simulink model "sm_car_Axle3_withDSD"  (R2022a)
settings: Solver=ode23t  StartTime=0.0  StopTime=40  MaxStep=0.4  RelTol=1e-3  AbsTol=1e-3  EnableMultiTasking=on
PreLoadFcn:
  | disp('Loading default data for 3-axle vehicle and 2-axle trailer')
  | if verLessThan('matlab', '9.11')
  |     load Vehicle_Axle3_008
  |     Vehicle = Vehicle_Axle3_008;
  |     load Trailer_Axle2_000
  |     Trailer = Trailer_Axle2_000;
  | else
  |     load Vehicle_Axle3_019
  |     Vehicle = Vehicle_Axle3_019;
  |     load Trailer_Axle2_022
  |     Trailer = Trailer_Axle2_022;
  | end
  | 
  | disp('Turning off MFEval warnings...')
  | disp('Solver:CoeffChecks:Eyk -- OFF')
  | disp('Solver:Limits:Exceeded -- OFF')
  | disp('Solver:CoeffChecks:Et -- OFF')
  | disp('Solver:CoeffChecks:Exa -- OFF')
  | 
  | warning('off','Solver:CoeffChecks:Eyk')
  | warning('off','Solver:Limits:Exceeded')
  | warning('off','Solver:CoeffChecks:Et')
  | warning('off','Solver:CoeffChecks:Exa')
  | %warning('off','Solver:Radius:NegativeRho')
  | 
  | % Due to usability issue in Repeating Sequence block
  | warning('off','Simulink:Masking:Invalid');
  | 
  | % Eliminate unnecessary warnings in inactive variants
  | % Warnings generated only if you click through inactive variant
  | warning('off','MATLAB:nonExistentField');
  | warning('off','Simulink:Parameters:BlkParamUndefined');
PostLoadFcn:
  | set_param([bdroot '/Vehicle'],'popup_trailer','On')
  | warning('off','sm:sli:setup:compile:LocalSolverNotSupported')
  | sm_car_config_maneuver(bdroot,'WOT Braking');
  | sm_car_config_vehicle(bdroot,false);
  | sm_car_config_logging(bdroot);
InitFcn:
  | sm_car_config_camera;
  | Vehicle = sm_car_vehcfg_checkConfig(Vehicle);
StartFcn:
  | sm_car_check_tire_model(bdroot);
  | tic;
StopFcn:
  | Elapsed_Sim_Time = toc;
  | % disp(['Elapsed Sim Time = ' num2str(Elapsed_Sim_Time)]);
values from neighbouring files (symbols this model uses):
  scenario = drivingScenario    [AEB_PedestrianChild_Nearside_50width_overrun.m]
undefined symbols (not defined in the file or in its folder): Maneuver, SimParams, X, Y, Z
libraries: simulink x16, Tire_Utilities x7, sm_lib x6, sm_car_DSD_lib x3, World_Config_Utilities x2, Maneuver_Get_Pose x2, Vehicle_Visualization x2, drivingscenarioandsensors x1, Camera_Frame_Definitions x1, Brake_Control x1, Driveline_Control_Axle2_None x1, Power_Control_Axle2_FixedRatio x1
(part 2 of 3)

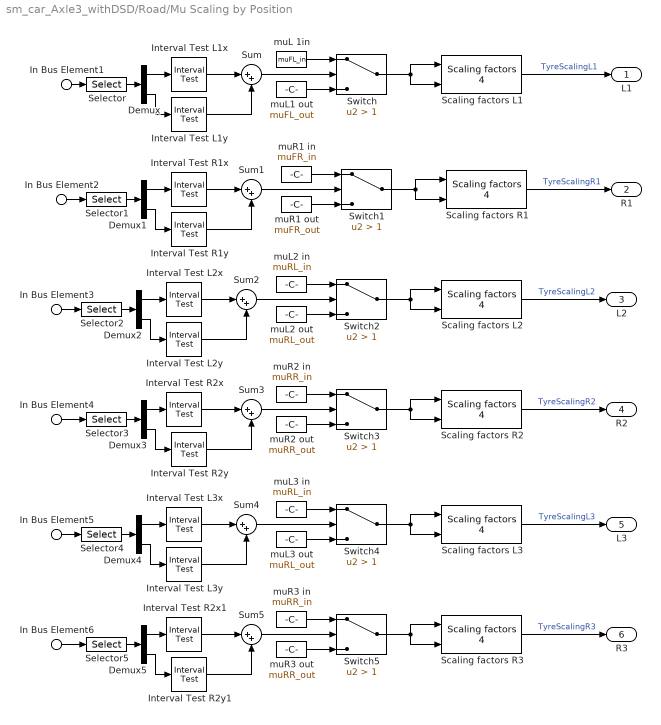
== system sm_car_Axle3_withDSD/Road/Mu Scaling by Position ==
  In Bus Element1 : Inport  PortName=Chassis  Element=WhlL1.xyz
  In Bus Element2 : Inport  PortName=Chassis  Element=WhlR1.xyz
  In Bus Element3 : Inport  PortName=Chassis  Element=WhlL2.xyz
  In Bus Element4 : Inport  PortName=Chassis  Element=WhlR2.xyz
  In Bus Element5 : Inport  PortName=Chassis  Element=WhlL3.xyz
  In Bus Element6 : Inport  PortName=Chassis  Element=WhlR3.xyz
  Demux{,1..5} (6 alike) : Demux  Outputs=2
  Interval Test L1x : simulink/Logic and Bit Operations/Interval Test  IntervalClosedRight=on  uplimit=intvX_FL_end  IntervalClosedLeft=on  lowlimit=intvX_FL_start  OutDataTypeStr=uint8
  Interval Test L1y : simulink/Logic and Bit Operations/Interval Test  IntervalClosedRight=on  uplimit=intvY_FL_end  IntervalClosedLeft=on  lowlimit=intvY_FL_start  OutDataTypeStr=uint8
  Interval Test L2x : simulink/Logic and Bit Operations/Interval Test  IntervalClosedRight=on  uplimit=intvX_RL_end  IntervalClosedLeft=on  lowlimit=intvX_RL_start  OutDataTypeStr=uint8
  Interval Test L2y : simulink/Logic and Bit Operations/Interval Test  IntervalClosedRight=on  uplimit=intvY_RL_end  IntervalClosedLeft=on  lowlimit=intvY_RL_start  OutDataTypeStr=uint8
  Interval Test L3x : simulink/Logic and Bit Operations/Interval Test  IntervalClosedRight=on  uplimit=intvX_RL_end  IntervalClosedLeft=on  lowlimit=intvX_RL_start  OutDataTypeStr=uint8
  Interval Test L3y : simulink/Logic and Bit Operations/Interval Test  IntervalClosedRight=on  uplimit=intvY_RL_end  IntervalClosedLeft=on  lowlimit=intvY_RL_start  OutDataTypeStr=uint8
  Interval Test R1x : simulink/Logic and Bit Operations/Interval Test  IntervalClosedRight=on  uplimit=intvX_FR_end  IntervalClosedLeft=on  lowlimit=intvX_FR_start  OutDataTypeStr=uint8
  Interval Test R1y : simulink/Logic and Bit Operations/Interval Test  IntervalClosedRight=on  uplimit=intvY_FR_end  IntervalClosedLeft=on  lowlimit=intvY_FR_start  OutDataTypeStr=uint8
  Interval Test R2x : simulink/Logic and Bit Operations/Interval Test  IntervalClosedRight=on  uplimit=intvX_RR_end  IntervalClosedLeft=on  lowlimit=intvX_RR_start  OutDataTypeStr=uint8
  Interval Test R2x1 : simulink/Logic and Bit Operations/Interval Test  IntervalClosedRight=on  uplimit=intvX_RR_end  IntervalClosedLeft=on  lowlimit=intvX_RR_start  OutDataTypeStr=uint8
  Interval Test R2y : simulink/Logic and Bit Operations/Interval Test  IntervalClosedRight=on  uplimit=intvY_RR_end  IntervalClosedLeft=on  lowlimit=intvY_RR_start  OutDataTypeStr=uint8
  Interval Test R2y1 : simulink/Logic and Bit Operations/Interval Test  IntervalClosedRight=on  uplimit=intvY_RR_end  IntervalClosedLeft=on  lowlimit=intvY_RR_start  OutDataTypeStr=uint8
  Scaling factors L1 : Tire_Utilities/Scaling factors 4  LKX=1  LKY=1  LKYC=1  LTR=1  LKZC=1
  Scaling factors L2 : Tire_Utilities/Scaling factors 4  LKX=1  LKY=1  LKYC=1  LTR=1  LKZC=1
  Scaling factors L3 : Tire_Utilities/Scaling factors 4  LKX=1  LKY=1  LKYC=1  LTR=1  LKZC=1
  Scaling factors R1 : Tire_Utilities/Scaling factors 4  LKX=1  LKY=1  LKYC=1  LTR=1  LKZC=1
  Scaling factors R2 : Tire_Utilities/Scaling factors 4  LKX=1  LKY=1  LKYC=1  LTR=1  LKZC=1
  Scaling factors R3 : Tire_Utilities/Scaling factors 4  LKX=1  LKY=1  LKYC=1  LTR=1  LKZC=1
  Selector{,1..5} (6 alike) : Selector  InputPortWidth=3  IndexOptions=Index vector (dialog)  Indices=[1 2]  OutputSizes=1
  Sum{,1..5} (6 alike) : Sum  Inputs=|++
  Switch : Switch  Criteria=u2 > Threshold  Threshold=1  ZeroCross=off  SaturateOnIntegerOverflow=off  InputSameDT=off
  Switch{1..5} (5 alike) : Switch  Criteria=u2 > Threshold  Threshold=1  SaturateOnIntegerOverflow=off  InputSameDT=off
  muL 1in : Constant  Value=muFL_in
  muL1 out : Constant  Value=muFL_out
  muL2 in : Constant  Value=muRL_in
  muL2 out : Constant  Value=muRL_out
  muL3 in : Constant  Value=muRL_in
  muL3 out : Constant  Value=muRL_out
  muR1 in : Constant  Value=muFR_in
  muR1 out : Constant  Value=muFR_out
  muR2 in : Constant  Value=muRR_in
  muR2 out : Constant  Value=muRR_out
  muR3 in : Constant  Value=muRR_in
  muR3 out : Constant  Value=muRR_out
  L1 : Outport  VectorParamsAs1DForOutWhenUnconnected=off
  R1 : Outport  Port=2  VectorParamsAs1DForOutWhenUnconnected=off
  L2 : Outport  Port=3  VectorParamsAs1DForOutWhenUnconnected=off
  R2 : Outport  Port=4  VectorParamsAs1DForOutWhenUnconnected=off
  L3 : Outport  Port=5  VectorParamsAs1DForOutWhenUnconnected=off
  R3 : Outport  Port=6  VectorParamsAs1DForOutWhenUnconnected=off
  wires:
  Demux/1 -> Interval Test L1x/1
  Interval Test R2x/1 -> Sum3/1
  Demux3/2 -> Interval Test R2y/1
  Demux3/1 -> Interval Test R2x/1
  Sum3/1 -> Switch3/2
  Selector3/1 -> Demux3/1
  In Bus Element4/1 -> Selector3/1
  Interval Test R2y/1 -> Sum3/2
  Demux2/2 -> Interval Test L2y/1
  Selector2/1 -> Demux2/1
  Demux2/1 -> Interval Test L2x/1
  Interval Test L2y/1 -> Sum2/2
  Sum2/1 -> Switch2/2
  In Bus Element3/1 -> Selector2/1
  Interval Test L2x/1 -> Sum2/1
  Interval Test R1y/1 -> Sum1/2
  Selector1/1 -> Demux1/1
  Demux1/2 -> Interval Test R1y/1
  Sum1/1 -> Switch1/2
  Demux1/1 -> Interval Test R1x/1
  Interval Test R1x/1 -> Sum1/1
  Interval Test L1x/1 -> Sum/1
  Interval Test L1y/1 -> Sum/2
  Sum/1 -> Switch/2
  Demux/2 -> Interval Test L1y/1
  Selector/1 -> Demux/1
  muR2 out/1 -> Switch3/3
  muR2 in/1 -> Switch3/1
  Switch3/1 -> Scaling factors R2/2, Scaling factors R2/1
  Scaling factors R2/1 -> R2/1  "TyreScalingR2"
  Scaling factors L2/1 -> L2/1  "TyreScalingL2"
  Switch2/1 -> Scaling factors L2/1, Scaling factors L2/2
  muL2 in/1 -> Switch2/1
  muL2 out/1 -> Switch2/3
  muR1 out/1 -> Switch1/3
  In Bus Element2/1 -> Selector1/1
  muR1 in/1 -> Switch1/1
  Switch1/1 -> Scaling factors R1/2, Scaling factors R1/1
  Scaling factors R1/1 -> R1/1  "TyreScalingR1"
  Scaling factors L1/1 -> L1/1  "TyreScalingL1"
  Switch/1 -> Scaling factors L1/1, Scaling factors L1/2
  muL1 out/1 -> Switch/3
  muL 1in/1 -> Switch/1
  In Bus Element1/1 -> Selector/1
  muL3 out/1 -> Switch4/3
  Switch4/1 -> Scaling factors L3/2, Scaling factors L3/1
  Scaling factors L3/1 -> L3/1  "TyreScalingL3"
  Scaling factors R3/1 -> R3/1  "TyreScalingR3"
  Switch5/1 -> Scaling factors R3/1, Scaling factors R3/2
  muR3 in/1 -> Switch5/1
  muR3 out/1 -> Switch5/3
  Interval Test L3x/1 -> Sum4/1
  In Bus Element5/1 -> Selector4/1
  Sum4/1 -> Switch4/2
  Interval Test L3y/1 -> Sum4/2
  Demux4/1 -> Interval Test L3x/1
  Selector4/1 -> Demux4/1
  Demux4/2 -> Interval Test L3y/1
  Interval Test R2y1/1 -> Sum5/2
  In Bus Element6/1 -> Selector5/1
  Selector5/1 -> Demux5/1
  Sum5/1 -> Switch5/2
  Demux5/1 -> Interval Test R2x1/1
  Demux5/2 -> Interval Test R2y1/1
  Interval Test R2x1/1 -> Sum5/1
  muL3 in/1 -> Switch4/1

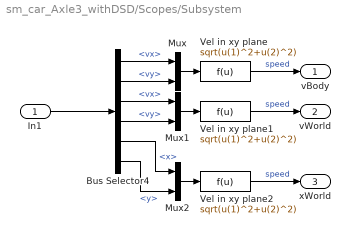
== system sm_car_Axle3_withDSD/Scopes/Subsystem ==
  In1 : Inport
  Bus Selector4 : BusSelector  OutputSignals=Chassis.Body.CG.vx,Chassis.Body.CG.vy,World.vx,World.vy,World.x,World.y
  Mux : Mux  Inputs=2
  Mux1 : Mux  Inputs=2
  Mux2 : Mux  Inputs=2
  Vel in xy plane : Fcn  Expr=sqrt(u(1)^2+u(2)^2)
  Vel in xy plane1 : Fcn  Expr=sqrt(u(1)^2+u(2)^2)
  Vel in xy plane2 : Fcn  Expr=sqrt(u(1)^2+u(2)^2)
  vBody : Outport  VectorParamsAs1DForOutWhenUnconnected=off
  vWorld : Outport  Port=2  VectorParamsAs1DForOutWhenUnconnected=off
  xWorld : Outport  Port=3  VectorParamsAs1DForOutWhenUnconnected=off
  wires:
  Bus Selector4/3 -> Mux1/1  "<vx>"
  Bus Selector4/4 -> Mux1/2  "<vy>"
  Bus Selector4/1 -> Mux/1  "<vx>"
  Vel in xy plane1/1 -> vWorld/1  "speed"
  In1/1 -> Bus Selector4/1
  Mux1/1 -> Vel in xy plane1/1
  Mux/1 -> Vel in xy plane/1
  Vel in xy plane/1 -> vBody/1  "speed"
  Bus Selector4/2 -> Mux/2  "<vy>"
  Mux2/1 -> Vel in xy plane2/1
  Bus Selector4/6 -> Mux2/2  "<y>"
  Bus Selector4/5 -> Mux2/1  "<x>"
  Vel in xy plane2/1 -> xWorld/1  "speed"

== system sm_car_Axle3_withDSD/Vehicle/Hitch ==
  Off : Subsystem  VariantControl=Off
  On : Subsystem  VariantControl=On
  " F" : PMIOPort  Side=Right
  " B" : PMIOPort  Port=2  Side=Left

== system sm_car_Axle3_withDSD/Vehicle/Vehicle Constraint ==
  No Constraint : Subsystem  VariantControl=NoConstraint
  No Yaw : Subsystem  VariantControl=NoYaw
  F : PMIOPort  Side=Right
  B : PMIOPort  Port=2  Side=Left

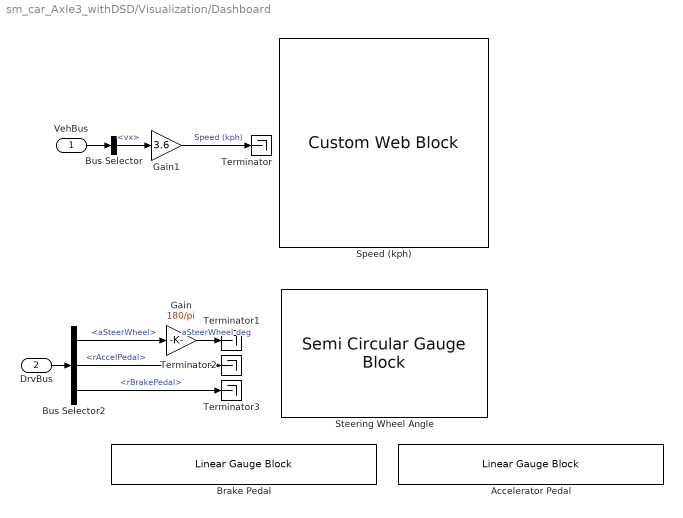
== system sm_car_Axle3_withDSD/Visualization/Dashboard ==
  VehBus : Inport
  DrvBus : Inport  Port=2
  Accelerator Pedal : LinearGaugeBlock  LabelPosition=Hide  ScaleMax=1
  Brake Pedal : LinearGaugeBlock  ScaleMax=1
  Bus Selector : BusSelector  OutputSignals=Chassis.Body.CG.vx
  Bus Selector2 : BusSelector  OutputSignals=aSteerWheel,rAccelPedal,rBrakePedal
  Gain : Gain  Gain=180/pi
  Gain1 : Gain  Gain=3.6
  Speed (kph) : CustomWebBlock  LabelPosition=Hide  ShowInitialText=on  Configuration="{\"components\":[{\"name\":\"CircularScaleComponent\",\"settings\":{\"bounds\":{\"max\":150,\"min\":0,\"tickInterval\":\"auto\"},\"direction\":\"cw\",\"flipLimits\":0,\"innerRadius\":0.46396628518311167,\"internalTickHeightScaleFactor\":1,\"labelColor\":[250,245,200],\"labelFont\":{\"font\":\"Arial\",\"fontSize\":12},\"labelRadius\":0.3050476634899135,\"labelTransparency\":1,\"minorTickHeightScaleFactor\":0.2,\"needleImage\":{\"size\":[1890,567],\"src\":\"data:image\\/svg+xml;base64,PD94bWwgdmVyc2lvbj0iMS4wIiBlbmNvZGluZz0iVVRGLTgiIHN0YW5kYWxvbmU9Im5vIj8+CjxzdmcKICAgeG1sbnM6ZGM9Imh0dHA6Ly9wdXJsLm9yZy9kYy9lbGVtZW50cy8xLjEvIgogICB4bWxuczpjYz0iaHR0cDovL2NyZWF0aXZlY29tbW9ucy5vcmcvbnMjIgogICB4bWxuczpyZGY9Imh0dHA6Ly93d3cudzMub3JnLzE5OTkvMDIvMjItcmRmLXN5bnRheC1ucyMiCiAgIHhtbG5zOnN2Zz0iaHR0cDovL3d3dy53My5vcmcvMjAwMC9zdmciCiAgIHhtbG5zPSJodHRwOi8vd3d3LnczLm9yZy8yMDAwL3N2ZyIKICAgeG1sbnM6 ...(+4096 chars)\"},\"needleOffset\":[0.09689320773631488,0],\"needleOrientation\":-45,\"needleRotation\":-180,\"needleSize\":{\"height\":0.0899722643265781,\"width\":0.2837586797992078},\"outerRadius\":0.6228849068763098,\"position\":[0,0,1,1],\"referencePoint\":\"auto\",\"scaleAngle\":299.999999999988,\"scaleAngleOffset\":119.46147497096791,\"scaleColors\":[],\"scaleColorsSize\":0.2,\"scaleDirection\":\"CW\",\"scalePosition\":[0,0,1,1],\"showLabels\":1,\"showMinorTicks\":1,\"showSpanLine\":1,\"showTicks\":1,\"tickColor\":[250,245,200],\"tickTransparency\":1,\"valueBarColor\":[23,89,176],\"valueBarPosition\":[0,0,1,1],\"valueBarSize\":0.2,\"valueBarTransparency\":1}},{\"name\":\"BackgroundImageComponent\",\"settings\":{\"image\":{\"size\":[0,0],\"src\":\"data:image\\/svg+xml;base64,PD94bWwgdmVyc2lvbj0iMS4wIiBlbmNvZGluZz0iVVRGLTgiIHN0YW5kYWxvbmU9Im5vIj8+CjwhLS0gR2VuZXJhdG9yOiBBZG9iZSBJbGx1c3RyYXRvciAxOS4yLjEsIFNWRyBFeHBvcnQgUGx1Zy1JbiAuIFNWRyBWZXJzaW9uOiA2LjAwIEJ1aWxkIDApICAtLT4KCjxzdmcKICAgeG1sbnM6ZGM9Imh0dHA6Ly9wdXJsLm9yZy9kYy9lbGVtZW50cy8xLjEvIgogICB4bWxuczpjYz0iaHR0cDovL2NyZWF0aXZlY29tbW9ucy5vcmcvbnMjIgogICB4bWxuczpyZGY9Imh0dHA6Ly93d3cudzMub3JnLzE5OTkvMDIvMjItcmRmLXN5bnRh ...(+9660 chars)\",\"srcOrientation\":\"horizontal\"},\"position\":[0,0,1,1],\"scaleMode\":\"0\"}},{\"name\":\"ForegroundImageComponent\",\"settings\":{\"image\":{\"size\":[0,0],\"src\":\"default\",\"srcOrientation\":[]},\"isForeground\":1,\"position\":[0,0,1,1],\"scaleMode\":\"0\"}}],\"settings\":{\"BindingType\":\"signal\",\"backgroundOffset\":0.14,\"backgroundOpacity\":1,\"fixedAspectRatio\":\"on\",\"orientation\":\"horizontal\",\"showBackgroundColor\":0,\"version\":\"R2022a\"},\"type\":\"CircularGauge\"}"
  Steering Wheel Angle : SemiCircularGaugeBlock  LabelPosition=Hide  ScaleMin=-80  ScaleMax=80  TickInterval=20
  Terminator{,1..3} (4 alike) : Terminator
  wires:
  VehBus/1 -> Bus Selector/1
  DrvBus/1 -> Bus Selector2/1
  Bus Selector/1 -> Gain1/1  "<vx>"
  Gain/1 -> Terminator1/1  "aSteerWheel deg"
  Bus Selector2/3 -> Terminator3/1  "<rBrakePedal>"
  Bus Selector2/1 -> Gain/1  "<aSteerWheel>"
  Bus Selector2/2 -> Terminator2/1  "<rAccelPedal>"
  Gain1/1 -> Terminator/1  "Speed (kph)"

== system sm_car_Axle3_withDSD/Visualization/Unreal ==
  "xyz " : Inport
  "rpy " : Inport  Port=2
  "ws " : Inport  Port=3
  "aCamber " : Inport  Port=4
  "aSteerWheel " : Inport  Port=5
  Animation Off : Subsystem  VariantControl=Off
  Animation On : Subsystem  VariantControl=On

== system sm_car_Axle3_withDSD/Driver/Closed Loop/Driver Override ==
  In : Inport
  None : Subsystem  VariantControl=None
  Override : Subsystem  VariantControl=Override
  DrvBus : Outport

== system sm_car_Axle3_withDSD/Driver/Closed Loop/Scopes ==
  <vx> : Inport
  Ref : Inport  Port=2
  CurPose : Inport  Port=3
  DrvBus : Inport  Port=4
  Bus Selector : BusSelector  OutputSignals=vTarget
  Bus Selector1 : BusSelector  OutputSignals=aSteerWheel,rAccelPedal,rBrakePedal
  Compare vx to Target : Scope  NumInputPorts=2
  RefPose : Scope
  Scope1 : Scope  NumInputPorts=3
  wires:
  DrvBus/1 -> Bus Selector1/1
  Bus Selector1/1 -> Scope1/1  "<aSteerWheel>"
  Bus Selector1/2 -> Scope1/2  "<rAccelPedal>"
  <vx>/1 -> Compare vx to Target/1
  Bus Selector1/3 -> Scope1/3  "<rBrakePedal>"
  CurPose/1 -> RefPose/1
  Bus Selector/1 -> Compare vx to Target/2  "<vTarget>"
  Ref/1 -> Bus Selector/1

== system sm_car_Axle3_withDSD/Driver/Interactive/Pace Car ==
  "VehBus " : Inport
  None : Subsystem  VariantControl=None
  Show : Subsystem  VariantControl=Show

== system sm_car_Axle3_withDSD/Vehicle/Hitch/Off ==
  Reference Frame : sm_lib/Frames and Transforms/Reference Frame
  F : PMIOPort  Side=Right
  B : PMIOPort  Port=2  Side=Left
  connections:
  B/RConn1 -- Reference Frame/RConn1

== system sm_car_Axle3_withDSD/Vehicle/Hitch/On ==
  Gimbal Joint : sm_lib/Joints/Gimbal Joint  JointMode=Normal  SenseConstraintForce=off  SenseConstraintForceX=off  SenseConstraintForceY=off  SenseConstraintForceZ=off  SenseConstraintTorque=off  SenseConstraintTorqueX=off  SenseConstraintTorqueY=off  SenseConstraintTorqueZ=off  SenseTotalForce=off  SenseTotalForceX=off  SenseTotalForceY=off  SenseTotalForceZ=off  SenseTotalTorque=off  SenseTotalTorqueX=off  SenseTotalTorqueY=off  SenseTotalTorqueZ=off  CompositeWrenchDir=FollowerOnBase  CompositeWrenchFrame=BaseFrame  RxEquilibriumPosition=0  RxEquilibriumPositionUnits=deg  RxSpringStiffness=1000  RxSpringStiffnessUnits=N*m/deg  RxDampingCoefficient=10  RxDampingCoefficientUnits=N*m/(deg/s)  RxTorqueActuationMode=NoTorque  RxMotionActuationMode=ComputedMotion  RxSensePosition=off  RxSenseVelocity=off  RxSenseAcceleration=off  RxSenseTorqueForce=off  RxSenseLowerLimitTorqueForce=off  RxSenseUpperLimitTorqueForce=off  RxLowerLimitSpecify=off  RxLowerLimitBound=-90  RxLowerLimitBoundUnits=deg  RxLowerLimitStiffness=1e4  RxLowerLimitStiffnessUnits=N*m/deg  RxLowerLimitDamping=10  RxLowerLimitDampingUnits=N*m/(deg/s)  RxLowerLimitTransitionRegionWidth=0.1  RxLowerLimitTransitionRegionWidthUnits=deg  RxUpperLimitSpecify=off  RxUpperLimitBound=90  RxUpperLimitBoundUnits=deg  RxUpperLimitStiffness=1e4  RxUpperLimitStiffnessUnits=N*m/deg  RxUpperLimitDamping=10  RxUpperLimitDampingUnits=N*m/(deg/s)  RxUpperLimitTransitionRegionWidth=0.1  RxUpperLimitTransitionRegionWidthUnits=deg  RxPositionTargetSpecify=on  RxPositionTargetPriority=High  RxPositionTargetValue=0  RxPositionTargetValueUnits=deg  RxVelocityTargetSpecify=off  RxVelocityTargetPriority=High  RxVelocityTargetValue=0  RxVelocityTargetValueUnits=deg/s  RyEquilibriumPosition=0  RyEquilibriumPositionUnits=deg  RySpringStiffness=1000  RySpringStiffnessUnits=N*m/deg  RyDampingCoefficient=10  RyDampingCoefficientUnits=N*m/(deg/s)  RyTorqueActuationMode=NoTorque  RyMotionActuationMode=ComputedMotion  RySensePosition=off  RySenseVelocity=off  RySenseAcceleration=off  RySenseTorqueForce=off  RySenseLowerLimitTorqueForce=off  RySenseUpperLimitTorqueForce=off  RyLowerLimitSpecify=off  RyLowerLimitBound=-90  RyLowerLimitBoundUnits=deg  RyLowerLimitStiffness=1e4  RyLowerLimitStiffnessUnits=N*m/deg  RyLowerLimitDamping=10  RyLowerLimitDampingUnits=N*m/(deg/s)  RyLowerLimitTransitionRegionWidth=0.1  RyLowerLimitTransitionRegionWidthUnits=deg  RyUpperLimitSpecify=off  RyUpperLimitBound=90  RyUpperLimitBoundUnits=deg  RyUpperLimitStiffness=1e4  RyUpperLimitStiffnessUnits=N*m/deg  RyUpperLimitDamping=10  RyUpperLimitDampingUnits=N*m/(deg/s)  RyUpperLimitTransitionRegionWidth=0.1  RyUpperLimitTransitionRegionWidthUnits=deg  RyPositionTargetSpecify=on  RyPositionTargetPriority=High  RyPositionTargetValue=0  RyPositionTargetValueUnits=deg  RyVelocityTargetSpecify=off  RyVelocityTargetPriority=High  RyVelocityTargetValue=0  RyVelocityTargetValueUnits=deg/s  RzEquilibriumPosition=0  RzEquilibriumPositionUnits=deg  RzSpringStiffness=0  RzSpringStiffnessUnits=N*m/deg  RzDampingCoefficient=0  RzDampingCoefficientUnits=N*m/(deg/s)  RzTorqueActuationMode=NoTorque  RzMotionActuationMode=ComputedMotion  RzSensePosition=off  RzSenseVelocity=off  RzSenseAcceleration=off  RzSenseTorqueForce=off  RzSenseLowerLimitTorqueForce=off  RzSenseUpperLimitTorqueForce=off  RzLowerLimitSpecify=off  RzLowerLimitBound=-90  RzLowerLimitBoundUnits=deg  RzLowerLimitStiffness=1e4  RzLowerLimitStiffnessUnits=N*m/deg  RzLowerLimitDamping=10  RzLowerLimitDampingUnits=N*m/(deg/s)  RzLowerLimitTransitionRegionWidth=0.1  RzLowerLimitTransitionRegionWidthUnits=deg  RzUpperLimitSpecify=off  RzUpperLimitBound=90  RzUpperLimitBoundUnits=deg  RzUpperLimitStiffness=1e4  RzUpperLimitStiffnessUnits=N*m/deg  RzUpperLimitDamping=10  RzUpperLimitDampingUnits=N*m/(deg/s)  RzUpperLimitTransitionRegionWidth=0.1  RzUpperLimitTransitionRegionWidthUnits=deg  RzPositionTargetSpecify=on  RzPositionTargetPriority=High  RzPositionTargetValue=0  RzPositionTargetValueUnits=deg  RzVelocityTargetSpecify=off  RzVelocityTargetPriority=High  RzVelocityTargetValue=0  RzVelocityTargetValueUnits=deg/s
  Spherical Joint : sm_lib/Joints/Spherical Joint  Commented=on  JointMode=Normal  SenseConstraintForce=off  SenseConstraintForceX=off  SenseConstraintForceY=off  SenseConstraintForceZ=off  SenseConstraintTorque=off  SenseConstraintTorqueX=off  SenseConstraintTorqueY=off  SenseConstraintTorqueZ=off  SenseTotalForce=off  SenseTotalForceX=off  SenseTotalForceY=off  SenseTotalForceZ=off  SenseTotalTorque=off  SenseTotalTorqueX=off  SenseTotalTorqueY=off  SenseTotalTorqueZ=off  CompositeWrenchDir=FollowerOnBase  CompositeWrenchFrame=BaseFrame  DefPosRotationMethod=None  DefPosRotationAngleUnits=deg  DefPosRotationStandardAxis=+Z  DefPosRotationAngle=0.0  DefPosRotationArbitraryAxis=[0 0 1]  DefPosFollAlignAxisA=+X  DefPosBaseAlignAxisA=+Y  DefPosFollAlignAxisB=+Y  DefPosBaseAlignAxisB=+Z  DefPosRotationSequenceAxes=FollowerAxes  DefPosRotationSequence=XYX  DefPosRotationSequenceAngles=[0 0 0]  DefPosRotationSequenceAnglesUnits=deg  DefPosRotationMatrix=[1 0 0; 0 1 0; 0 0 1]  EqPosRotationMethod=None  EqPosRotationAngleUnits=deg  EqPosRotationStandardAxis=+Z  EqPosRotationAngle=0.0  EqPosRotationArbitraryAxis=[0 0 1]  EqPosFollAlignAxisA=+X  EqPosBaseAlignAxisA=+Y  EqPosFollAlignAxisB=+Y  EqPosBaseAlignAxisB=+Z  EqPosRotationSequenceAxes=FollowerAxes  EqPosRotationSequence=XYX  EqPosRotationSequenceAngles=[0 0 0]  EqPosRotationSequenceAnglesUnits=deg  EqPosRotationMatrix=[1 0 0; 0 1 0; 0 0 1]  SpringStiffness=100  SpringStiffnessUnits=N*m/deg  DampingCoefficient=0.1  DampingCoefficientUnits=N*m/(deg/s)  ActuateTorqueX=off  ActuateTorqueY=off  ActuateTorqueZ=off  ActuateTorque=off  TorqueActuationMode=NoTorque  MotionActuationMode=ComputedMotion  ActuationFrame=BaseFrame  SensePosition=off  SenseVelocityX=off  SenseVelocityY=off  SenseVelocityZ=off  SenseVelocity=off  SenseAccelerationX=off  SenseAccelerationY=off  SenseAccelerationZ=off  SenseAcceleration=off  SenseTorqueX=off  SenseTorqueY=off  SenseTorqueZ=off  SenseTorqueForce=off  SenseLowerLimitTorqueMag=off  SenseUpperLimitTorqueMag=off  SensingFrame=BaseFrame  LowerLimitSpecify=off  LowerLimitBound=15  LowerLimitBoundUnits=deg  LowerLimitStiffness=1e4  LowerLimitStiffnessUnits=N*m/deg  LowerLimitDamping=10  LowerLimitDampingUnits=N*m/(deg/s)  LowerLimitTransitionRegionWidth=0.1  LowerLimitTransitionRegionWidthUnits=deg  UpperLimitSpecify=off  UpperLimitBound=45  UpperLimitBoundUnits=deg  UpperLimitStiffness=1e4  UpperLimitStiffnessUnits=N*m/deg  UpperLimitDamping=10  UpperLimitDampingUnits=N*m/(deg/s)  UpperLimitTransitionRegionWidth=0.1  UpperLimitTransitionRegionWidthUnits=deg  PositionTargetRotationMethod=None  PositionTargetRotationAngleUnits=deg  PositionTargetRotationStandardAxis=+Z  PositionTargetRotationAngle=0.0  PositionTargetRotationArbitraryAxis=[0 0 1]  PositionTargetFollAlignAxisA=+X  PositionTargetBaseAlignAxisA=+Y  PositionTargetFollAlignAxisB=+Y  PositionTargetBaseAlignAxisB=+Z  PositionTargetRotationSequenceAxes=FollowerAxes  PositionTargetRotationSequence=XYX  PositionTargetRotationSequenceAngles=[0 0 0]  PositionTargetRotationSequenceAnglesUnits=deg  PositionTargetRotationMatrix=[1 0 0; 0 1 0; 0 0 1]  PositionTargetSpecify=on  PositionTargetPriority=High  VelocityTargetValue=[0 0 0]  VelocityTargetValueUnits=deg/s  VelocityTargetSpecify=off  VelocityTargetPriority=High  VelocityTargetInFollowerFrame=on
  F : PMIOPort  Side=Right
  B : PMIOPort  Port=2  Side=Left
  connections:
  Gimbal Joint/LConn1 -- B/RConn1
  Gimbal Joint/RConn1 -- F/RConn1

== system sm_car_Axle3_withDSD/Vehicle/Vehicle Constraint/No Constraint ==
  F : PMIOPort  Side=Right
  B : PMIOPort  Port=2  Side=Left

== system sm_car_Axle3_withDSD/Vehicle/Vehicle Constraint/No Yaw ==
  Cartesian Joint : sm_lib/Joints/Cartesian Joint  JointMode=Normal  SenseConstraintForce=off  SenseConstraintForceX=off  SenseConstraintForceY=off  SenseConstraintForceZ=off  SenseConstraintTorque=off  SenseConstraintTorqueX=off  SenseConstraintTorqueY=off  SenseConstraintTorqueZ=off  SenseTotalForce=off  SenseTotalForceX=off  SenseTotalForceY=off  SenseTotalForceZ=off  SenseTotalTorque=off  SenseTotalTorqueX=off  SenseTotalTorqueY=off  SenseTotalTorqueZ=off  CompositeWrenchDir=FollowerOnBase  CompositeWrenchFrame=BaseFrame  PxEquilibriumPosition=0  PxEquilibriumPositionUnits=m  PxSpringStiffness=0  PxSpringStiffnessUnits=N/m  PxDampingCoefficient=0  PxDampingCoefficientUnits=N/(m/s)  PxTorqueActuationMode=NoTorque  PxMotionActuationMode=ComputedMotion  PxSensePosition=off  PxSenseVelocity=off  PxSenseAcceleration=off  PxSenseTorqueForce=off  PxSenseLowerLimitTorqueForce=off  PxSenseUpperLimitTorqueForce=off  PxLowerLimitSpecify=off  PxLowerLimitBound=-1  PxLowerLimitBoundUnits=m  PxLowerLimitStiffness=1e6  PxLowerLimitStiffnessUnits=N/m  PxLowerLimitDamping=1e3  PxLowerLimitDampingUnits=N/(m/s)  PxLowerLimitTransitionRegionWidth=1e-4  PxLowerLimitTransitionRegionWidthUnits=m  PxUpperLimitSpecify=off  PxUpperLimitBound=1  PxUpperLimitBoundUnits=m  PxUpperLimitStiffness=1e6  PxUpperLimitStiffnessUnits=N/m  PxUpperLimitDamping=1e3  PxUpperLimitDampingUnits=N/(m/s)  PxUpperLimitTransitionRegionWidth=1e-4  PxUpperLimitTransitionRegionWidthUnits=m  PxPositionTargetSpecify=off  PxPositionTargetPriority=High  PxPositionTargetValue=0  PxPositionTargetValueUnits=m  PxVelocityTargetSpecify=off  PxVelocityTargetPriority=High  PxVelocityTargetValue=0  PxVelocityTargetValueUnits=m/s  PyEquilibriumPosition=0  PyEquilibriumPositionUnits=m  PySpringStiffness=0  PySpringStiffnessUnits=N/m  PyDampingCoefficient=0  PyDampingCoefficientUnits=N/(m/s)  PyTorqueActuationMode=NoTorque  PyMotionActuationMode=ComputedMotion  PySensePosition=off  PySenseVelocity=off  PySenseAcceleration=off  PySenseTorqueForce=off  PySenseLowerLimitTorqueForce=off  PySenseUpperLimitTorqueForce=off  PyLowerLimitSpecify=off  PyLowerLimitBound=-1  PyLowerLimitBoundUnits=m  PyLowerLimitStiffness=1e6  PyLowerLimitStiffnessUnits=N/m  PyLowerLimitDamping=1e3  PyLowerLimitDampingUnits=N/(m/s)  PyLowerLimitTransitionRegionWidth=1e-4  PyLowerLimitTransitionRegionWidthUnits=m  PyUpperLimitSpecify=off  PyUpperLimitBound=1  PyUpperLimitBoundUnits=m  PyUpperLimitStiffness=1e6  PyUpperLimitStiffnessUnits=N/m  PyUpperLimitDamping=1e3  PyUpperLimitDampingUnits=N/(m/s)  PyUpperLimitTransitionRegionWidth=1e-4  PyUpperLimitTransitionRegionWidthUnits=m  PyPositionTargetSpecify=off  PyPositionTargetPriority=High  PyPositionTargetValue=0  PyPositionTargetValueUnits=m  PyVelocityTargetSpecify=off  PyVelocityTargetPriority=High  PyVelocityTargetValue=0  PyVelocityTargetValueUnits=m/s  PzEquilibriumPosition=0  PzEquilibriumPositionUnits=m  PzSpringStiffness=0  PzSpringStiffnessUnits=N/m  PzDampingCoefficient=0  PzDampingCoefficientUnits=N/(m/s)  PzTorqueActuationMode=NoTorque  PzMotionActuationMode=ComputedMotion  PzSensePosition=off  PzSenseVelocity=off  PzSenseAcceleration=off  PzSenseTorqueForce=off  PzSenseLowerLimitTorqueForce=off  PzSenseUpperLimitTorqueForce=off  PzLowerLimitSpecify=off  PzLowerLimitBound=-1  PzLowerLimitBoundUnits=m  PzLowerLimitStiffness=1e6  PzLowerLimitStiffnessUnits=N/m  PzLowerLimitDamping=1e3  PzLowerLimitDampingUnits=N/(m/s)  PzLowerLimitTransitionRegionWidth=1e-4  PzLowerLimitTransitionRegionWidthUnits=m  PzUpperLimitSpecify=off  PzUpperLimitBound=1  PzUpperLimitBoundUnits=m  PzUpperLimitStiffness=1e6  PzUpperLimitStiffnessUnits=N/m  PzUpperLimitDamping=1e3  PzUpperLimitDampingUnits=N/(m/s)  PzUpperLimitTransitionRegionWidth=1e-4  PzUpperLimitTransitionRegionWidthUnits=m  PzPositionTargetSpecify=off  PzPositionTargetPriority=High  PzPositionTargetValue=0  PzPositionTargetValueUnits=m  PzVelocityTargetSpecify=off  PzVelocityTargetPriority=High  PzVelocityTargetValue=0  PzVelocityTargetValueUnits=m/s
  Universal Joint : sm_lib/Joints/Universal Joint  JointMode=Normal  SenseConstraintForce=off  SenseConstraintForceX=off  SenseConstraintForceY=off  SenseConstraintForceZ=off  SenseConstraintTorque=off  SenseConstraintTorqueX=off  SenseConstraintTorqueY=off  SenseConstraintTorqueZ=off  SenseTotalForce=off  SenseTotalForceX=off  SenseTotalForceY=off  SenseTotalForceZ=off  SenseTotalTorque=off  SenseTotalTorqueX=off  SenseTotalTorqueY=off  SenseTotalTorqueZ=off  CompositeWrenchDir=FollowerOnBase  CompositeWrenchFrame=BaseFrame  RxEquilibriumPosition=0  RxEquilibriumPositionUnits=deg  RxSpringStiffness=0  RxSpringStiffnessUnits=N*m/deg  RxDampingCoefficient=0  RxDampingCoefficientUnits=N*m/(deg/s)  RxTorqueActuationMode=NoTorque  RxMotionActuationMode=ComputedMotion  RxSensePosition=off  RxSenseVelocity=off  RxSenseAcceleration=off  RxSenseTorqueForce=off  RxSenseLowerLimitTorqueForce=off  RxSenseUpperLimitTorqueForce=off  RxLowerLimitSpecify=off  RxLowerLimitBound=-90  RxLowerLimitBoundUnits=deg  RxLowerLimitStiffness=1e4  RxLowerLimitStiffnessUnits=N*m/deg  RxLowerLimitDamping=10  RxLowerLimitDampingUnits=N*m/(deg/s)  RxLowerLimitTransitionRegionWidth=0.1  RxLowerLimitTransitionRegionWidthUnits=deg  RxUpperLimitSpecify=off  RxUpperLimitBound=90  RxUpperLimitBoundUnits=deg  RxUpperLimitStiffness=1e4  RxUpperLimitStiffnessUnits=N*m/deg  RxUpperLimitDamping=10  RxUpperLimitDampingUnits=N*m/(deg/s)  RxUpperLimitTransitionRegionWidth=0.1  RxUpperLimitTransitionRegionWidthUnits=deg  RxPositionTargetSpecify=off  RxPositionTargetPriority=High  RxPositionTargetValue=0  RxPositionTargetValueUnits=deg  RxVelocityTargetSpecify=off  RxVelocityTargetPriority=High  RxVelocityTargetValue=0  RxVelocityTargetValueUnits=deg/s  RyEquilibriumPosition=0  RyEquilibriumPositionUnits=deg  RySpringStiffness=0  RySpringStiffnessUnits=N*m/deg  RyDampingCoefficient=0  RyDampingCoefficientUnits=N*m/(deg/s)  RyTorqueActuationMode=NoTorque  RyMotionActuationMode=ComputedMotion  RySensePosition=off  RySenseVelocity=off  RySenseAcceleration=off  RySenseTorqueForce=off  RySenseLowerLimitTorqueForce=off  RySenseUpperLimitTorqueForce=off  RyLowerLimitSpecify=off  RyLowerLimitBound=-90  RyLowerLimitBoundUnits=deg  RyLowerLimitStiffness=1e4  RyLowerLimitStiffnessUnits=N*m/deg  RyLowerLimitDamping=10  RyLowerLimitDampingUnits=N*m/(deg/s)  RyLowerLimitTransitionRegionWidth=0.1  RyLowerLimitTransitionRegionWidthUnits=deg  RyUpperLimitSpecify=off  RyUpperLimitBound=90  RyUpperLimitBoundUnits=deg  RyUpperLimitStiffness=1e4  RyUpperLimitStiffnessUnits=N*m/deg  RyUpperLimitDamping=10  RyUpperLimitDampingUnits=N*m/(deg/s)  RyUpperLimitTransitionRegionWidth=0.1  RyUpperLimitTransitionRegionWidthUnits=deg  RyPositionTargetSpecify=off  RyPositionTargetPriority=High  RyPositionTargetValue=0  RyPositionTargetValueUnits=deg  RyVelocityTargetSpecify=off  RyVelocityTargetPriority=High  RyVelocityTargetValue=0  RyVelocityTargetValueUnits=deg/s
  F : PMIOPort  Side=Right
  B : PMIOPort  Port=2  Side=Left
  connections:
  Cartesian Joint/LConn1 -- B/RConn1
  Cartesian Joint/RConn1 -- Universal Joint/LConn1
  Universal Joint/RConn1 -- F/RConn1

== system sm_car_Axle3_withDSD/Visualization/Unreal/Animation Off ==
  xyz : Inport
  rpy : Inport  Port=2
  ws : Inport  Port=3
  aCamber : Inport  Port=4
  aSteerWheel : Inport  Port=5
  Terminator{,1..4} (5 alike) : Terminator
  wires:
  rpy/1 -> Terminator1/1
  aSteerWheel/1 -> Terminator4/1
  aCamber/1 -> Terminator3/1
  xyz/1 -> Terminator/1
  ws/1 -> Terminator2/1

== system sm_car_Axle3_withDSD/Visualization/Unreal/Animation On ==
  xyz : Inport
  rpy : Inport  Port=2
  ws : Inport  Port=3
  aCamber : Inport  Port=4
  aSteerWheel : Inport  Port=5
  Transform Data for Uneal : Vehicle_Visualization/Transform Data for Unreal  SystemSampleTime=-1  VariantActivationTime=update diagram  Latency=0  AutoFrameSizeCalculation=off
  Unreal Animation : Subsystem
  wires:
  Transform Data for Uneal/2 -> Unreal Animation/2(Rotation)  "Unreal_Rotation"
  Transform Data for Uneal/1 -> Unreal Animation/1(Translation)  "Unreal_Translation"
  ws/1 -> Transform Data for Uneal/3
  xyz/1 -> Transform Data for Uneal/1
  aCamber/1 -> Transform Data for Uneal/4
  aSteerWheel/1 -> Transform Data for Uneal/5
  rpy/1 -> Transform Data for Uneal/2

== system sm_car_Axle3_withDSD/Driver/Closed Loop/Driver Override/None ==
  In : Inport
  DrvBus : Outport
  wires:
  In/1 -> DrvBus/1

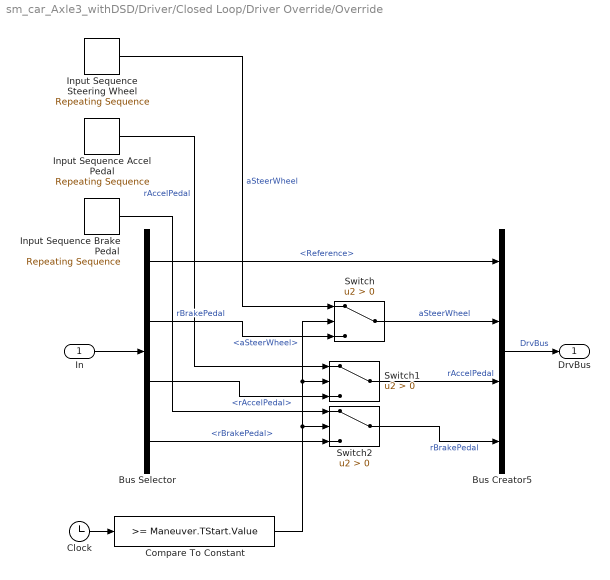
== system sm_car_Axle3_withDSD/Driver/Closed Loop/Driver Override/Override ==
  In : Inport
  Bus Creator5 : BusCreator  Inputs=4
  Bus Selector : BusSelector  OutputSignals=Reference,aSteerWheel,rAccelPedal,rBrakePedal
  Clock : Clock
  Compare To Constant : simulink/Logic and Bit Operations/Compare To Constant  relop=>=  const=Maneuver.TStart.Value  OutDataTypeStr=boolean
  Input Sequence Accel Pedal : simulink/Sources/Repeating Sequence  rep_seq_t=Maneuver.Accel.t.Value  rep_seq_y=Maneuver.Accel.rPedal.Value
  Input Sequence Brake Pedal : simulink/Sources/Repeating Sequence  rep_seq_t=Maneuver.Brake.t.Value  rep_seq_y=Maneuver.Brake.rPedal.Value
  "Input Sequence Steering Wheel " : simulink/Sources/Repeating Sequence  rep_seq_t=Maneuver.Steer.t.Value  rep_seq_y=Maneuver.Steer.aWheel.Value
  Switch : Switch  Criteria=u2 > Threshold  SaturateOnIntegerOverflow=off  InputSameDT=off
  Switch1 : Switch  Criteria=u2 > Threshold  SaturateOnIntegerOverflow=off  InputSameDT=off
  Switch2 : Switch  Criteria=u2 > Threshold  SaturateOnIntegerOverflow=off  InputSameDT=off
  DrvBus : Outport
  wires:
  In/1 -> Bus Selector/1
  Bus Creator5/1 -> DrvBus/1  "DrvBus"
  Bus Selector/2 -> Switch/3  "<aSteerWheel>"
  Switch/1 -> Bus Creator5/2  "aSteerWheel"
  Bus Selector/1 -> Bus Creator5/1  "<Reference>"
  Bus Selector/3 -> Switch1/3  "<rAccelPedal>"
  Switch1/1 -> Bus Creator5/3  "rAccelPedal"
  Bus Selector/4 -> Switch2/3  "<rBrakePedal>"
  Clock/1 -> Compare To Constant/1
  Compare To Constant/1 -> Switch2/2, Switch1/2, Switch/2
  Switch2/1 -> Bus Creator5/4  "rBrakePedal"
  "Input Sequence Steering Wheel "/1 -> Switch/1  "aSteerWheel"
  Input Sequence Accel Pedal/1 -> Switch1/1  "rAccelPedal"
  Input Sequence Brake Pedal/1 -> Switch2/1  "rBrakePedal"

== system sm_car_Axle3_withDSD/Driver/Interactive/Pace Car/None ==
  "VehBus " : Inport
  Terminator : Terminator
  wires:
  "VehBus "/1 -> Terminator/1

== system sm_car_Axle3_withDSD/Driver/Interactive/Pace Car/Show ==
  "VehBus " : Inport
  Maneuver : Maneuver_Get_Pose/Maneuver  Maneuver=Maneuver  popup_window=No
  Terminator{,1..3} (4 alike) : Terminator
  wires:
  ? -> Terminator3/1
  Maneuver/3 -> Terminator2/1
  Maneuver/2 -> Terminator1/1
  Maneuver/1 -> Terminator/1
  "VehBus "/1 -> Maneuver/1
